simulink model "scheme_L2"  (R2025a)
settings: Solver=ode4  StartTime=0  StopTime=10  FixedStep=0.001  RelTol=1e-3
settings Model: Creator=ekaterinaberezneva  LastModifiedBy=ekaterinaberezneva

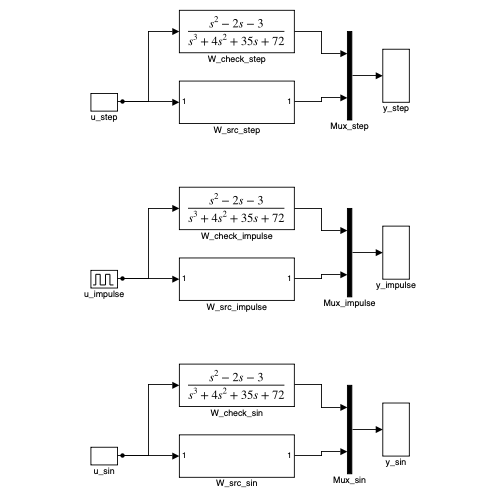
[thumbnail: Simulink's stored preview of the top-level diagram]
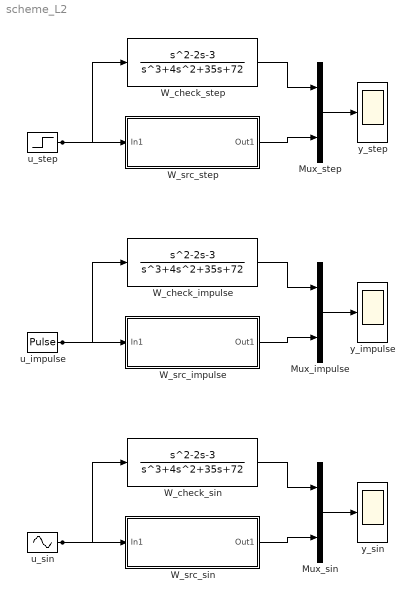
== system scheme_L2 ==
  Mux_impulse : Mux  Inputs=2
  Mux_sin : Mux  Inputs=2
  Mux_step : Mux  Inputs=2
  W_check_impulse : TransferFcn  Numerator=[1 -2 -3]  Denominator=[1 4 35 72]
  W_check_sin : TransferFcn  Numerator=[1 -2 -3]  Denominator=[1 4 35 72]
  W_check_step : TransferFcn  Numerator=[1 -2 -3]  Denominator=[1 4 35 72]
  W_src_impulse : Subsystem
  W_src_sin : Subsystem
  W_src_step : Subsystem
  u_impulse : DiscretePulseGenerator  PulseType=Time based  Amplitude=20  Period=20  PulseWidth=0.2  PhaseDelay=2
  u_sin : Sin  Frequency=3  SampleTime=0
  u_step : Step  SampleTime=0
  y_impulse : Scope
      settings: DataLoggingVariableName=y_impulse_log
  y_sin : Scope
      settings: DataLoggingVariableName=y_sin_log
  y_step : Scope
      settings: DataLoggingVariableName=y_step_log
  wires:
  u_step/1 -> W_src_step/1(In1), W_check_step/1
  u_impulse/1 -> W_src_impulse/1(In1), W_check_impulse/1
  u_sin/1 -> W_src_sin/1(In1), W_check_sin/1
  W_check_step/1 -> Mux_step/1
  W_src_step/1(Out1) -> Mux_step/2
  W_check_impulse/1 -> Mux_impulse/1
  W_src_impulse/1(Out1) -> Mux_impulse/2
  W_check_sin/1 -> Mux_sin/1
  W_src_sin/1(Out1) -> Mux_sin/2
  Mux_step/1 -> y_step/1
  Mux_impulse/1 -> y_impulse/1
  Mux_sin/1 -> y_sin/1

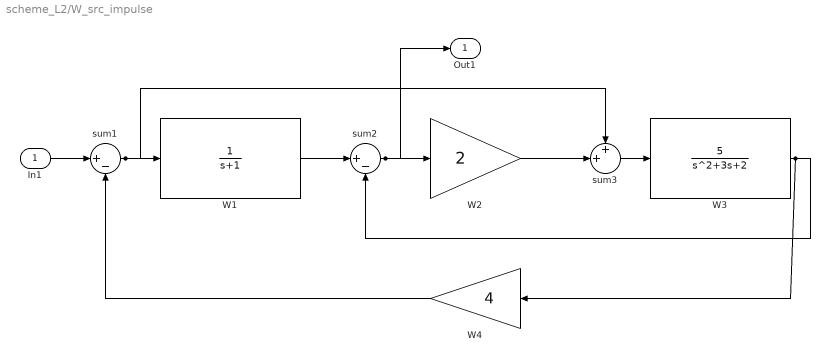
== system scheme_L2/W_src_impulse ==
  In1 : Inport
  W1 : TransferFcn  Denominator=[1 1]
  W2 : Gain  Gain=2
  W3 : TransferFcn  Numerator=[5]  Denominator=[1 3 2]
  W4 : Gain  Gain=4
  sum1 : Sum  Inputs=|+-
  sum2 : Sum  Inputs=|+-
  sum3 : Sum  Inputs=++|
  Out1 : Outport
  wires:
  W4/1 -> sum1/2
  W3/1 -> W4/1, sum2/2
  sum3/1 -> W3/1
  W2/1 -> sum3/2
  sum2/1 -> Out1/1, W2/1
  W1/1 -> sum2/1
  sum1/1 -> sum3/1, W1/1
  In1/1 -> sum1/1

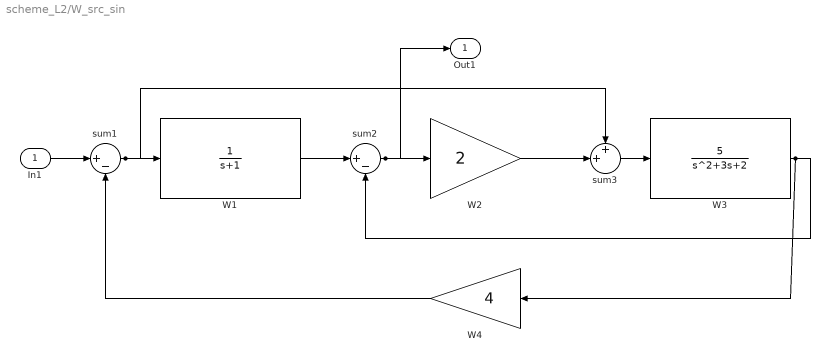
== system scheme_L2/W_src_sin ==
  In1 : Inport
  W1 : TransferFcn  Denominator=[1 1]
  W2 : Gain  Gain=2
  W3 : TransferFcn  Numerator=[5]  Denominator=[1 3 2]
  W4 : Gain  Gain=4
  sum1 : Sum  Inputs=|+-
  sum2 : Sum  Inputs=|+-
  sum3 : Sum  Inputs=++|
  Out1 : Outport
  wires:
  W4/1 -> sum1/2
  W3/1 -> W4/1, sum2/2
  sum3/1 -> W3/1
  W2/1 -> sum3/2
  sum2/1 -> Out1/1, W2/1
  W1/1 -> sum2/1
  sum1/1 -> sum3/1, W1/1
  In1/1 -> sum1/1

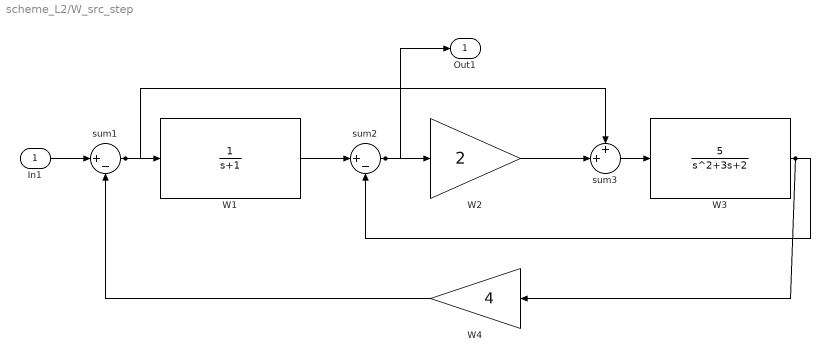
== system scheme_L2/W_src_step ==
  In1 : Inport
  W1 : TransferFcn  Denominator=[1 1]
  W2 : Gain  Gain=2
  W3 : TransferFcn  Numerator=[5]  Denominator=[1 3 2]
  W4 : Gain  Gain=4
  sum1 : Sum  Inputs=|+-
  sum2 : Sum  Inputs=|+-
  sum3 : Sum  Inputs=++|
  Out1 : Outport
  wires:
  In1/1 -> sum1/1
  sum1/1 -> W1/1, sum3/1
  W1/1 -> sum2/1
  sum2/1 -> W2/1, Out1/1
  W2/1 -> sum3/2
  sum3/1 -> W3/1
  W3/1 -> sum2/2, W4/1
  W4/1 -> sum1/2
